simulink model "CabinTempController_SIL_vs_MIL"  (R2015a)
settings: Solver=FixedStepDiscrete  StartTime=0.0  StopTime=10.0  FixedStep=0.01  RelTol=1e-3
libraries: simulink x2, pil_lib x1
settings Model: Creator=A.hegazy  LastModifiedBy=A.hegazy
settings DataIOCC: SaveFormat=Dataset
settings OptimizationCC: OptimizeModelRefInitCode=on  LifeSpan=1
settings HardwareCC: ProdBitPerPointer=64  ProdLongLongMode=on  ProdHWDeviceType=Generic->64-bit Embedded Processor (LLP64)  TargetBitPerLong=64  TargetBitPerPointer=64  TargetIntDivRoundTo=Zero  TargetEndianess=LittleEndian  TargetWordSize=64  TargetHWDeviceType=Intel->x86-64
settings RTWCC: SystemTargetFile=ert.tlc  TemplateMakefile=ert_default_tmf  Description=Embedded Coder  GenerateReport=on  PortableWordSizes=on  CreateSILPILBlock=SIL
settings CodeAppCC: IgnoreCustomStorageClasses=off
settings ERTTargetCC: ParMdlRefBuildCompliant=on  CompOptLevelCompliant=on  ConcurrentExecutionCompliant=on  ERTFirstTimeCompliant=on  SupportContinuousTime=off  SupportVariableSizeSignals=off  ModelStepFunctionPrototypeControlCompliant=on  CPPClassGenCompliant=on  InlinedParameterPlacement=Hierarchical  ERTCustomFileTemplate=example_file_process.tlc

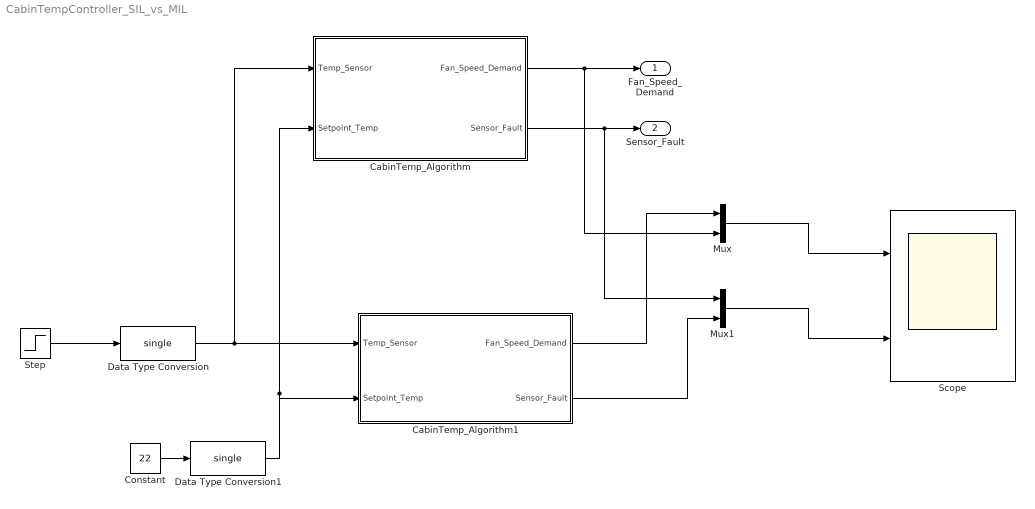
== system CabinTempController_SIL_vs_MIL ==
  CabinTemp_Algorithm : Subsystem  TreatAsAtomicUnit=on  SystemSampleTime=0.01
  CabinTemp_Algorithm1 : Subsystem  DialogController=pil_create_dialog  LoadFcn=|
      | try
      |    if ~strcmp(rtw.pil.getPILVersion, '6.8 (R2015a)_12')
      |       set_param(gcb, 'DialogController', '');
      |       set_param(gcb, 'DialogControllerArgs', '');
      |    end
      | catch e
      |       set_param(gcb, 'DialogController', '');
      |       set_param(gcb, 'DialogControllerArgs', '');
      | end
      mask help: PIL:pil:XILBlockMaskDesc
      mask Display: disp('SIL');
  Constant : Constant  Value=22  OutDataTypeStr=single
  Data Type Conversion : DataTypeConversion  OutDataTypeStr=single
  Data Type Conversion1 : DataTypeConversion  OutDataTypeStr=single
  Mux : Mux  Inputs=2
  Mux1 : Mux  Inputs=2
  Scope : Scope  NumInputPorts=2
      settings: YMin=-5~-5  YMax=5~5
  Step : Step  After=100  SampleTime=0
  Fan_Speed_Demand : Outport
  Sensor_Fault : Outport  Port=2
  wires:
  CabinTemp_Algorithm/1(Fan_Speed_Demand) -> Mux/2, Fan_Speed_Demand/1
  CabinTemp_Algorithm/2(Sensor_Fault) -> Mux1/1, Sensor_Fault/1
  CabinTemp_Algorithm1/1(Fan_Speed_Demand) -> Mux/1
  Mux/1 -> Scope/1
  CabinTemp_Algorithm1/2(Sensor_Fault) -> Mux1/2
  Mux1/1 -> Scope/2
  Step/1 -> Data Type Conversion/1
  Constant/1 -> Data Type Conversion1/1
  Data Type Conversion/1 -> CabinTemp_Algorithm1/1(Temp_Sensor), CabinTemp_Algorithm/1(Temp_Sensor)
  Data Type Conversion1/1 -> CabinTemp_Algorithm/2(Setpoint_Temp), CabinTemp_Algorithm1/2(Setpoint_Temp)

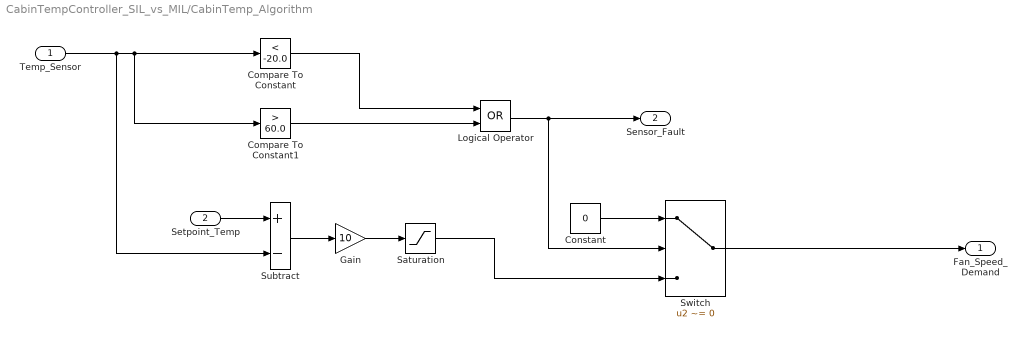
== system CabinTempController_SIL_vs_MIL/CabinTemp_Algorithm ==
  Temp_Sensor : Inport  OutDataTypeStr=single  SampleTime=0.01
  Setpoint_Temp : Inport  Port=2  OutDataTypeStr=single  SampleTime=0.01
  Compare To Constant : simulink/Logic and Bit Operations/Compare To Constant  relop=<  const=-20.0  OutDataTypeStr=boolean
  Compare To Constant1 : simulink/Logic and Bit Operations/Compare To Constant  relop=>  const=60.0  OutDataTypeStr=boolean
  Constant : Constant  Value=0  OutDataTypeStr=single
  Gain : Gain  Gain=10
  Logical Operator : Logic  Operator=OR  AllPortsSameDT=off  OutDataTypeStr=boolean
  Saturation : Saturate  UpperLimit=100  LowerLimit=0
  Subtract : Sum  Inputs=+-
  Switch : Switch  Criteria=u2 ~= 0
  Fan_Speed_Demand : Outport  OutDataTypeStr=single
  Sensor_Fault : Outport  Port=2  OutDataTypeStr=boolean
  wires:
  Temp_Sensor/1 -> Subtract/2, Compare To Constant1/1, Compare To Constant/1
  Compare To Constant/1 -> Logical Operator/1
  Compare To Constant1/1 -> Logical Operator/2
  Logical Operator/1 -> Switch/2, Sensor_Fault/1
  Setpoint_Temp/1 -> Subtract/1
  Subtract/1 -> Gain/1
  Gain/1 -> Saturation/1
  Constant/1 -> Switch/1
  Saturation/1 -> Switch/3
  Switch/1 -> Fan_Speed_Demand/1

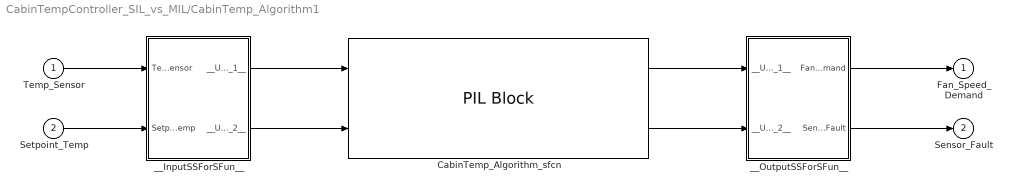
== system CabinTempController_SIL_vs_MIL/CabinTemp_Algorithm1 ==
  Temp_Sensor : Inport  OutDataTypeStr=single  SampleTime=0.01
  Setpoint_Temp : Inport  Port=2  OutDataTypeStr=single  SampleTime=0.01
  CabinTemp_Algorithm_sfcn : pil_lib/PIL Block  SimulationMode=SIL  IsTopModelPIL=off  CodeDir=C:\MBD_Project\CabinTemp_Algorithm_ert_rtw  ConfigName=Software-in-the-Loop (SIL)
  __InputSSForSFun__ : Subsystem
  __OutputSSForSFun__ : Subsystem
  Fan_Speed_Demand : Outport  OutDataTypeStr=single
  Sensor_Fault : Outport  Port=2  OutDataTypeStr=boolean
  wires:
  Temp_Sensor/1 -> __InputSSForSFun__/1(Temp_Sensor)
  Setpoint_Temp/1 -> __InputSSForSFun__/2(Setpoint_Temp)
  __InputSSForSFun__/1(__UniqueOutportName__1__) -> CabinTemp_Algorithm_sfcn/1
  __InputSSForSFun__/2(__UniqueOutportName__2__) -> CabinTemp_Algorithm_sfcn/2
  CabinTemp_Algorithm_sfcn/1 -> __OutputSSForSFun__/1(__UniqueInportName__1__)
  CabinTemp_Algorithm_sfcn/2 -> __OutputSSForSFun__/2(__UniqueInportName__2__)
  __OutputSSForSFun__/1(Fan_Speed_Demand) -> Fan_Speed_Demand/1
  __OutputSSForSFun__/2(Sensor_Fault) -> Sensor_Fault/1

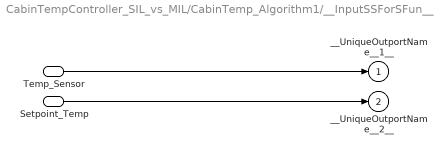
== system CabinTempController_SIL_vs_MIL/CabinTemp_Algorithm1/__InputSSForSFun__ ==
  Temp_Sensor : Inport  OutDataTypeStr=single  SampleTime=0.01
  Setpoint_Temp : Inport  Port=2  OutDataTypeStr=single  SampleTime=0.01
  __UniqueOutportName__1__ : Outport
  __UniqueOutportName__2__ : Outport  Port=2
  wires:
  Temp_Sensor/1 -> __UniqueOutportName__1__/1
  Setpoint_Temp/1 -> __UniqueOutportName__2__/1

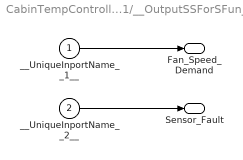
== system CabinTempController_SIL_vs_MIL/CabinTemp_Algorithm1/__OutputSSForSFun__ ==
  __UniqueInportName__1__ : Inport
  __UniqueInportName__2__ : Inport  Port=2
  Fan_Speed_Demand : Outport  OutDataTypeStr=single
  Sensor_Fault : Outport  Port=2  OutDataTypeStr=boolean
  wires:
  __UniqueInportName__1__/1 -> Fan_Speed_Demand/1
  __UniqueInportName__2__/1 -> Sensor_Fault/1
